simulink library "joystick_lib"  (R2018b)
settings: Solver=VariableStepAuto  StartTime=0.0  StopTime=10.0  RelTol=1e-3
undefined symbols (not defined in the file or in its folder): jystck
libraries: matlabinput_lib x1
settings Model: Creator=Ybeyer  LastModifiedBy=jonas
settings DebuggingCC: LibraryContextMissingDiagnostic=none
settings SFSimCC: SimUseLocalCustomCode=off
settings RTWCC: RTWUseLocalCustomCode=off
settings CodeAppCC: StateflowObjectComments=on

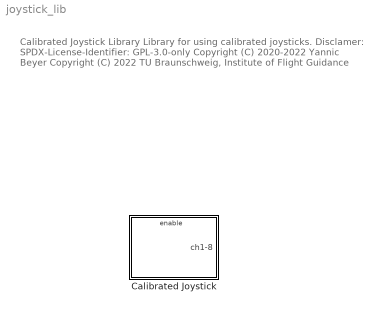
== system joystick_lib ==
  note: Calibrated Joystick Library
      |
      | Library for using calibrated joysticks.
      |
      | Disclamer:
      | SPDX-License-Identifier: GPL-3.0-only
      |
      | Copyright (C) 2020-2022 Yannic Beyer
      | Copyright (C) 2022 TU Braunschweig, Institute of Flight Guidance
  Calibrated Joystick : Subsystem  mask{jystck=jystck, joyid=1}
      mask prompts: jystck "joystick struct, see joystickLoadParams"; joyid "Joystick ID:"
      mask DialogControl DescGroupVar Prompt: Joystick
      mask DialogControl DescTextVar Prompt: This block should work on both Windows and Linux. By specification of the config you can use different types of joysticks.

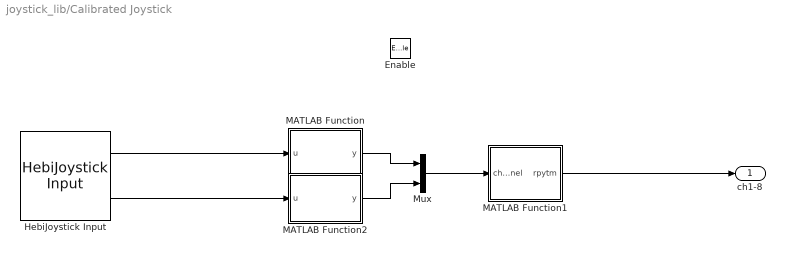
== system joystick_lib/Calibrated Joystick ==
  Enable : EnablePort
  HebiJoystick Input : matlabinput_lib/HebiJoystick Input  joyid=joyid  forcefeed=off
      settings: SourceProductName=MatlabInput
  MATLAB Function : MATLAB Function  TreatAsAtomicUnit=on
  MATLAB Function1 : MATLAB Function  TreatAsAtomicUnit=on
  MATLAB Function2 : MATLAB Function  TreatAsAtomicUnit=on
  Mux : Mux  Inputs=2
  ch1-8 : Outport
  wires:
  HebiJoystick Input/2 -> MATLAB Function2/1(u)
  MATLAB Function/1(y) -> Mux/1
  MATLAB Function1/1(rpytm) -> ch1-8/1
  HebiJoystick Input/1 -> MATLAB Function/1(u)
  MATLAB Function2/1(y) -> Mux/2
  Mux/1 -> MATLAB Function1/1(channel)

== matlab function joystick_lib/Calibrated Joystick/MATLAB Function1 ==
  data: channel input; rpytm output; jystck parameter
function rpytm = fcn( channel, jystck ) %#codegen
rpytm = joystickCh2Rpyt( channel, jystck );
end

== matlab function joystick_lib/Calibrated Joystick/MATLAB Function ==
  data: u input; y output
function y = fcn(u)

y = zeros(8,1);
y(1:length(u)) = u;

end

== matlab function joystick_lib/Calibrated Joystick/MATLAB Function2 ==
  data: u input; y output
function y = fcn(u)

y = zeros(8,1);
if length(u) > length(y)
    y(1:end) = u(1:8);
else
    y(1:length(u)) = u;
end

end
